simulink model "Lab1_3_2_2_Robust_AntiWindup"  (R2024b)
settings: Solver=ode5  StartTime=0.0  StopTime=3  FixedStep=1e-03  RelTol=1e-3
undefined symbols (not defined in the file): degs2rpm, delta_i, K_rob, Ki_rob, Kw, National_Instruments, Nu, Nx, PCI, rpm2rads, sens, wc, wc2
libraries: sldrtlib x2
settings Model: SimulationMode=external  ExtModeTrigDuration=45001  Creator=lenovo  LastModifiedBy=aboulenien
settings DataIOCC: ReturnWorkspaceOutputs=off
settings HardwareCC: ProdBitPerLong=64  ProdHWDeviceType=Intel->x86-64 (Linux 64)
settings RTWCC: Description=Simulink Desktop Real-Time  SystemTargetFile=sldrt.tlc  TemplateMakefile=sldrt.tmf  RTWCompilerOptimization=on
settings CodeAppCC: MaxIdLength=95
settings SimulinkDesktopRealTimeCC: TargetLibSuffix=_sldrt.a  TargetPreCompLibLocation=C:\Program Files\MATLAB\R2024b\toolbox\sldrt\lib\win64  ParMdlRefBuildCompliant=on

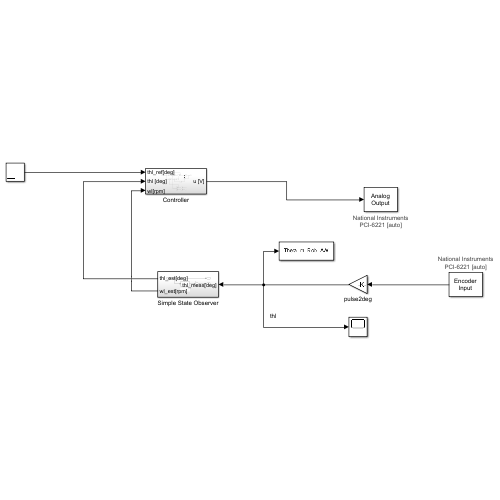
[thumbnail: Simulink's stored preview of the top-level diagram]
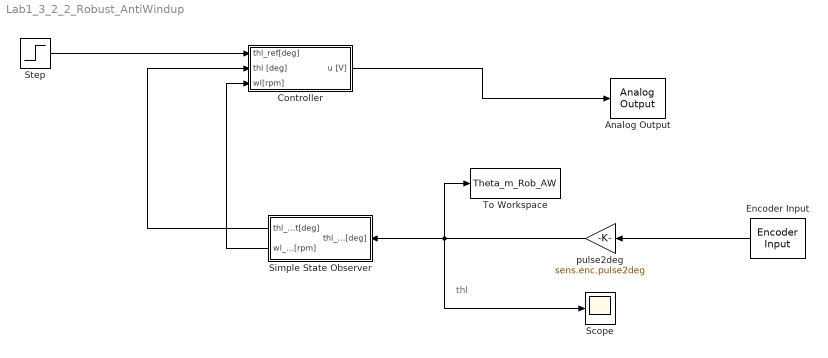
== system Lab1_3_2_2_Robust_AntiWindup ==
  note: thl
  Analog Output : sldrtlib/Analog Output  SampleTime=-1  MaxMissedTicks=10  ShowMissedTicks=off  YieldWhenWaiting=off  DrvName=National_Instruments/PCI-6221  DrvAddress=4294967295  DrvOptions=[0 0 0 2 0]  Channels=1  RangeMode=1  VoltRange=1  InitialValue=0  FinalValue=0
      settings: AttributesFormatString=National Instruments\nPCI-6221 [auto]
  Controller : Subsystem
  Encoder Input : sldrtlib/Encoder Input  SampleTime=-1  MaxMissedTicks=10  ShowMissedTicks=off  YieldWhenWaiting=off  DrvName=National_Instruments/PCI-6221  DrvAddress=4294967295  DrvOptions=[0 0 0 2 0]  Channels=1  QuadMode=3  IndexPulse=1  InputFilter=Inf  DataType=1
      settings: AttributesFormatString=National Instruments\nPCI-6221 [auto]
  Scope : Scope
  Simple State Observer : Subsystem
  Step : Step  After=40  SampleTime=0
  To Workspace : ToWorkspace  VariableName=Theta_m_Rob_AW  SaveFormat=Structure With Time  SampleTime=0.001
  pulse2deg : Gain  Gain=sens.enc.pulse2deg
  wires:
  Encoder Input/1 -> pulse2deg/1
  pulse2deg/1 -> Scope/1, To Workspace/1, Simple State Observer/1(thl_meas[deg])
  Controller/1(u [V]) -> Analog Output/1
  Step/1 -> Controller/1(thl_ref[deg])
  Simple State Observer/1(thl_est[deg]) -> Controller/2(thl [deg])
  Simple State Observer/2(wl_est[rpm]) -> Controller/3(wl[rpm])

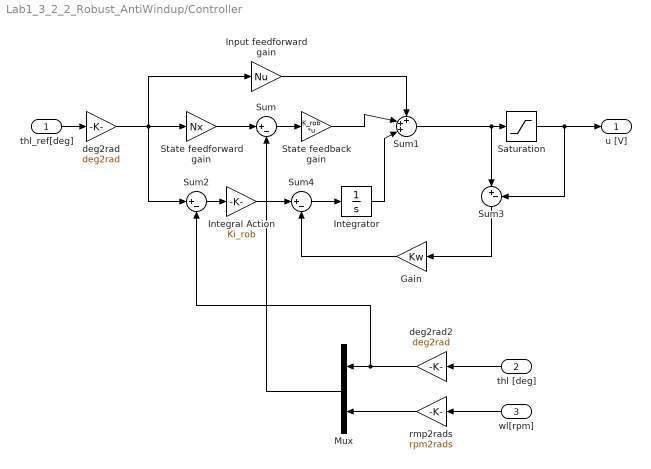
== system Lab1_3_2_2_Robust_AntiWindup/Controller ==
  thl_ref[deg] : Inport
  thl [deg] : Inport  Port=2
  wl[rpm] : Inport  Port=3
  Gain : Gain  Gain=Kw
  Input feedforward gain : Gain  Gain=Nu
  Integral Action : Gain  Gain=Ki_rob
  Integrator : Integrator
  Mux : Mux  Inputs=2
  Saturation : Saturate  UpperLimit=12  LowerLimit=-12
  State feedback gain : Gain  Gain=K_rob  Multiplication=Matrix(K*u)
  State feedforward gain : Gain  Gain=Nx
  Sum{,2..4} (4 alike) : Sum  Inputs=|+-
  Sum1 : Sum  Inputs=+++|
  deg2rad : Gain  Gain=deg2rad
  deg2rad2 : Gain  Gain=deg2rad
  rmp2rads : Gain  Gain=rpm2rads
  u [V] : Outport
  wires:
  thl_ref[deg]/1 -> deg2rad/1
  deg2rad/1 -> Sum2/1, Input feedforward gain/1, State feedforward gain/1
  State feedforward gain/1 -> Sum/1
  Sum/1 -> State feedback gain/1
  Saturation/1 -> Sum3/2, u [V]/1
  Mux/1 -> Sum/2
  deg2rad2/1 -> Sum2/2, Mux/1
  rmp2rads/1 -> Mux/2
  thl [deg]/1 -> deg2rad2/1
  wl[rpm]/1 -> rmp2rads/1
  Input feedforward gain/1 -> Sum1/1
  Sum1/1 -> Sum3/1, Saturation/1
  State feedback gain/1 -> Sum1/2
  Integrator/1 -> Sum1/3
  Sum2/1 -> Integral Action/1
  Sum3/1 -> Gain/1
  Gain/1 -> Sum4/2
  Integral Action/1 -> Sum4/1
  Sum4/1 -> Integrator/1

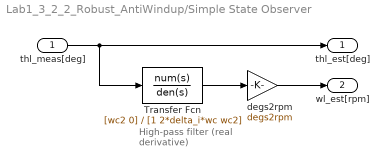
== system Lab1_3_2_2_Robust_AntiWindup/Simple State Observer ==
  note: High-pass filter
      | (real derivative)
  thl_meas[deg] : Inport
  Transfer Fcn : TransferFcn  Numerator=[wc2 0]  Denominator=[1 2*delta_i*wc wc2]
  degs2rpm : Gain  Gain=degs2rpm
  thl_est[deg] : Outport
  wl_est[rpm] : Outport  Port=2
  wires:
  thl_meas[deg]/1 -> Transfer Fcn/1, thl_est[deg]/1
  Transfer Fcn/1 -> degs2rpm/1
  degs2rpm/1 -> wl_est[rpm]/1
